simulink model "SpaceRobot"  (R2025b)
settings: Solver=ode4  StartTime=0.0  StopTime=8.5  FixedStep=0.01  RelTol=1e-5  AbsTol=1e-6
undefined symbols (not defined in the file or in its folder): d_safe, isdone_init, reward_init, Ts_agent, X, Y, Z
libraries: sm_lib x53, nesl_utility x34, rllib x1, sharedutil x1
(part 2 of 2)

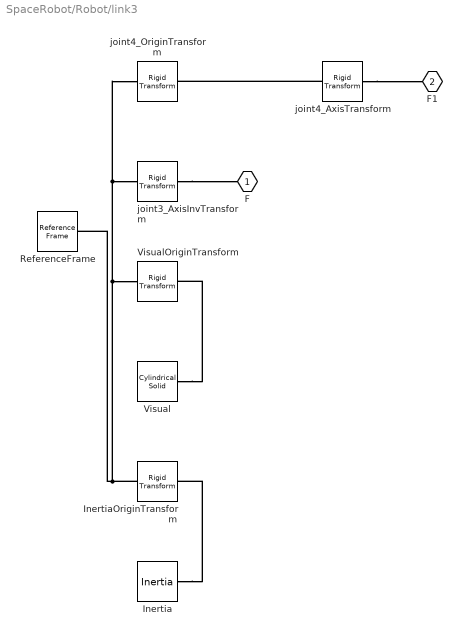
== system SpaceRobot/Robot/link3 ==
  Inertia : sm_lib/Body Elements/Inertia  InertiaType=Custom  Mass=1  MassUnits=kg  CenterOfMass=[0, 0, 0]  CenterOfMassUnits=m  MomentsOfInertia=[0.1, 0.1, 0.1]  MomentsOfInertiaUnits=kg*m^2  ProductsOfInertia=[0, 0, 0]  ProductsOfInertiaUnits=kg*m^2  GraphicType=None  MarkerShape=Inertia  MarkerSize=20  GraphicVisPropType=SimpleVisualProperties  GraphicDiffuseColor=[0.5 0.5 0.5]  GraphicOpacity=1  GraphicSpecularColor=[0.5 0.5 0.5 1.0]  GraphicAmbientColor=[0.15 0.15 0.15 1.0]  GraphicEmissiveColor=[0.0 0.0 0.0 1.0]  GraphicShininess=75
  InertiaOriginTransform : sm_lib/Frames and Transforms/Rigid Transform  RotationMethod=RotationSequence  FollAlignAxisA=+X  BaseAlignAxisA=+Y  FollAlignAxisB=+Y  BaseAlignAxisB=+Z  RotationStandardAxis=+Z  RotationAngle=0  RotationAngleUnits=deg  RotationArbitraryAxis=[0 0 1]  RotationSequenceAxes=BaseAxes  RotationSequence=XYZ  RotationSequenceAngles=[0, 0, 0]  RotationSequenceAnglesUnits=rad  RotationMatrix=[1 0 0;0 1 0;0 0 1]  Quaternion=[1 0 0 0]  TranslationMethod=Cartesian  TranslationCartesianOffset=[0.5, 0, 0]  TranslationCartesianOffsetUnits=m  TranslationStandardAxis=+Z  TranslationStandardOffset=0  TranslationStandardOffsetUnits=m  TranslationROffset=0  TranslationROffsetUnits=m  TranslationThetaOffset=0  TranslationThetaOffsetUnits=deg  TranslationZOffset=0  TranslationZOffsetUnits=m
  ReferenceFrame : sm_lib/Frames and Transforms/Reference Frame
  Visual : sm_lib/Body Elements/Cylindrical Solid  CylinderRadius=0.05  CylinderRadiusUnits=m  CylinderLength=1  CylinderLengthUnits=m  ExportEntireGeometry=off  InertiaType=Custom  BasedOnType=Density  Density=1000  DensityUnits=kg/m^3  Mass=1  MassUnits=kg  CenterOfMass=[0, 0, 0]  CenterOfMassUnits=m  MomentsOfInertia=[0.1, 0.1, 0.1]  MomentsOfInertiaUnits=kg*m^2  ProductsOfInertia=[0, 0, 0]  ProductsOfInertiaUnits=kg*m^2  GraphicType=FromGeometry  MarkerShape=Sphere  MarkerSize=10  GraphicVisPropType=SimpleVisualProperties  GraphicDiffuseColor=[0.7, 0.7, 0.7]  GraphicOpacity=1  GraphicSpecularColor=[0.5 0.5 0.5 1.0]  GraphicAmbientColor=[0.15 0.15 0.15 1.0]  GraphicEmissiveColor=[0.0 0.0 0.0 1.0]  GraphicShininess=75  DoExposeReferenceFrame=on  SerializedFrames=<Frames/>
  VisualOriginTransform : sm_lib/Frames and Transforms/Rigid Transform  RotationMethod=RotationSequence  FollAlignAxisA=+X  BaseAlignAxisA=+Y  FollAlignAxisB=+Y  BaseAlignAxisB=+Z  RotationStandardAxis=+Z  RotationAngle=0  RotationAngleUnits=deg  RotationArbitraryAxis=[0 0 1]  RotationSequenceAxes=BaseAxes  RotationSequence=XYZ  RotationSequenceAngles=[0, 1.5708, 0]  RotationSequenceAnglesUnits=rad  RotationMatrix=[1 0 0;0 1 0;0 0 1]  Quaternion=[1 0 0 0]  TranslationMethod=Cartesian  TranslationCartesianOffset=[0.5, 0, 0]  TranslationCartesianOffsetUnits=m  TranslationStandardAxis=+Z  TranslationStandardOffset=0  TranslationStandardOffsetUnits=m  TranslationROffset=0  TranslationROffsetUnits=m  TranslationThetaOffset=0  TranslationThetaOffsetUnits=deg  TranslationZOffset=0  TranslationZOffsetUnits=m
  joint3_AxisInvTransform : sm_lib/Frames and Transforms/Rigid Transform  RotationMethod=ArbitraryAxis  FollAlignAxisA=+X  BaseAlignAxisA=+Y  FollAlignAxisB=+Y  BaseAlignAxisB=+Z  RotationStandardAxis=+Z  RotationAngle=0  RotationAngleUnits=rad  RotationArbitraryAxis=[1, 0, 0]  RotationSequenceAxes=FollowerAxes  RotationSequence=XYX  RotationSequenceAngles=[0 0 0]  RotationSequenceAnglesUnits=deg  RotationMatrix=[1 0 0;0 1 0;0 0 1]  Quaternion=[1 0 0 0]  TranslationMethod=Cartesian  TranslationCartesianOffset=[0, 0, 0]  TranslationCartesianOffsetUnits=m  TranslationStandardAxis=+Z  TranslationStandardOffset=0  TranslationStandardOffsetUnits=m  TranslationROffset=0  TranslationROffsetUnits=m  TranslationThetaOffset=0  TranslationThetaOffsetUnits=deg  TranslationZOffset=0  TranslationZOffsetUnits=m
  joint4_AxisTransform : sm_lib/Frames and Transforms/Rigid Transform  RotationMethod=ArbitraryAxis  FollAlignAxisA=+X  BaseAlignAxisA=+Y  FollAlignAxisB=+Y  BaseAlignAxisB=+Z  RotationStandardAxis=+Z  RotationAngle=0  RotationAngleUnits=rad  RotationArbitraryAxis=[1, 0, 0]  RotationSequenceAxes=FollowerAxes  RotationSequence=XYX  RotationSequenceAngles=[0 0 0]  RotationSequenceAnglesUnits=deg  RotationMatrix=[1 0 0;0 1 0;0 0 1]  Quaternion=[1 0 0 0]  TranslationMethod=Cartesian  TranslationCartesianOffset=[0, 0, 0]  TranslationCartesianOffsetUnits=m  TranslationStandardAxis=+Z  TranslationStandardOffset=0  TranslationStandardOffsetUnits=m  TranslationROffset=0  TranslationROffsetUnits=m  TranslationThetaOffset=0  TranslationThetaOffsetUnits=deg  TranslationZOffset=0  TranslationZOffsetUnits=m
  joint4_OriginTransform : sm_lib/Frames and Transforms/Rigid Transform  RotationMethod=RotationSequence  FollAlignAxisA=+X  BaseAlignAxisA=+Y  FollAlignAxisB=+Y  BaseAlignAxisB=+Z  RotationStandardAxis=+Z  RotationAngle=0  RotationAngleUnits=deg  RotationArbitraryAxis=[0 0 1]  RotationSequenceAxes=BaseAxes  RotationSequence=XYZ  RotationSequenceAngles=[0, 0, 0]  RotationSequenceAnglesUnits=rad  RotationMatrix=[1 0 0;0 1 0;0 0 1]  Quaternion=[1 0 0 0]  TranslationMethod=Cartesian  TranslationCartesianOffset=[1, 0, 0]  TranslationCartesianOffsetUnits=m  TranslationStandardAxis=+Z  TranslationStandardOffset=0  TranslationStandardOffsetUnits=m  TranslationROffset=0  TranslationROffsetUnits=m  TranslationThetaOffset=0  TranslationThetaOffsetUnits=deg  TranslationZOffset=0  TranslationZOffsetUnits=m
  F : PMIOPort  Side=Left
  F1 : PMIOPort  Port=2  Side=Right
  connections:
  Inertia/RConn1 -- InertiaOriginTransform/RConn1
  ReferenceFrame/RConn1 -- InertiaOriginTransform/LConn1 -- joint3_AxisInvTransform/LConn1 -- joint4_OriginTransform/LConn1 -- VisualOriginTransform/LConn1
  Visual/RConn1 -- VisualOriginTransform/RConn1
  joint3_AxisInvTransform/RConn1 -- F/RConn1
  joint4_AxisTransform/RConn1 -- F1/RConn1
  joint4_AxisTransform/LConn1 -- joint4_OriginTransform/RConn1

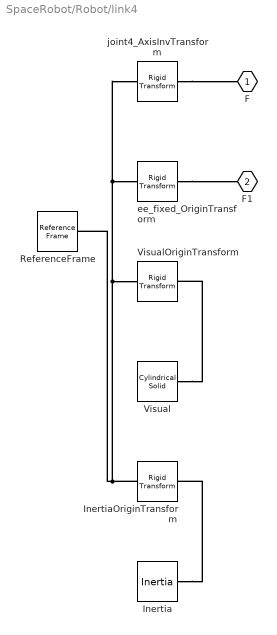
== system SpaceRobot/Robot/link4 ==
  Inertia : sm_lib/Body Elements/Inertia  InertiaType=Custom  Mass=1  MassUnits=kg  CenterOfMass=[0, 0, 0]  CenterOfMassUnits=m  MomentsOfInertia=[0.1, 0.1, 0.1]  MomentsOfInertiaUnits=kg*m^2  ProductsOfInertia=[0, 0, 0]  ProductsOfInertiaUnits=kg*m^2  GraphicType=None  MarkerShape=Inertia  MarkerSize=20  GraphicVisPropType=SimpleVisualProperties  GraphicDiffuseColor=[0.5 0.5 0.5]  GraphicOpacity=1  GraphicSpecularColor=[0.5 0.5 0.5 1.0]  GraphicAmbientColor=[0.15 0.15 0.15 1.0]  GraphicEmissiveColor=[0.0 0.0 0.0 1.0]  GraphicShininess=75
  InertiaOriginTransform : sm_lib/Frames and Transforms/Rigid Transform  RotationMethod=RotationSequence  FollAlignAxisA=+X  BaseAlignAxisA=+Y  FollAlignAxisB=+Y  BaseAlignAxisB=+Z  RotationStandardAxis=+Z  RotationAngle=0  RotationAngleUnits=deg  RotationArbitraryAxis=[0 0 1]  RotationSequenceAxes=BaseAxes  RotationSequence=XYZ  RotationSequenceAngles=[0, 0, 0]  RotationSequenceAnglesUnits=rad  RotationMatrix=[1 0 0;0 1 0;0 0 1]  Quaternion=[1 0 0 0]  TranslationMethod=Cartesian  TranslationCartesianOffset=[0.5, 0, 0]  TranslationCartesianOffsetUnits=m  TranslationStandardAxis=+Z  TranslationStandardOffset=0  TranslationStandardOffsetUnits=m  TranslationROffset=0  TranslationROffsetUnits=m  TranslationThetaOffset=0  TranslationThetaOffsetUnits=deg  TranslationZOffset=0  TranslationZOffsetUnits=m
  ReferenceFrame : sm_lib/Frames and Transforms/Reference Frame
  Visual : sm_lib/Body Elements/Cylindrical Solid  CylinderRadius=0.05  CylinderRadiusUnits=m  CylinderLength=1  CylinderLengthUnits=m  ExportEntireGeometry=off  InertiaType=Custom  BasedOnType=Density  Density=1000  DensityUnits=kg/m^3  Mass=1  MassUnits=kg  CenterOfMass=[0, 0, 0]  CenterOfMassUnits=m  MomentsOfInertia=[0.1, 0.1, 0.1]  MomentsOfInertiaUnits=kg*m^2  ProductsOfInertia=[0, 0, 0]  ProductsOfInertiaUnits=kg*m^2  GraphicType=FromGeometry  MarkerShape=Sphere  MarkerSize=10  GraphicVisPropType=SimpleVisualProperties  GraphicDiffuseColor=[0.8, 0.8, 0.8]  GraphicOpacity=1  GraphicSpecularColor=[0.5 0.5 0.5 1.0]  GraphicAmbientColor=[0.15 0.15 0.15 1.0]  GraphicEmissiveColor=[0.0 0.0 0.0 1.0]  GraphicShininess=75  DoExposeReferenceFrame=on  SerializedFrames=<Frames/>
  VisualOriginTransform : sm_lib/Frames and Transforms/Rigid Transform  RotationMethod=RotationSequence  FollAlignAxisA=+X  BaseAlignAxisA=+Y  FollAlignAxisB=+Y  BaseAlignAxisB=+Z  RotationStandardAxis=+Z  RotationAngle=0  RotationAngleUnits=deg  RotationArbitraryAxis=[0 0 1]  RotationSequenceAxes=BaseAxes  RotationSequence=XYZ  RotationSequenceAngles=[0, 1.5708, 0]  RotationSequenceAnglesUnits=rad  RotationMatrix=[1 0 0;0 1 0;0 0 1]  Quaternion=[1 0 0 0]  TranslationMethod=Cartesian  TranslationCartesianOffset=[0.5, 0, 0]  TranslationCartesianOffsetUnits=m  TranslationStandardAxis=+Z  TranslationStandardOffset=0  TranslationStandardOffsetUnits=m  TranslationROffset=0  TranslationROffsetUnits=m  TranslationThetaOffset=0  TranslationThetaOffsetUnits=deg  TranslationZOffset=0  TranslationZOffsetUnits=m
  ee_fixed_OriginTransform : sm_lib/Frames and Transforms/Rigid Transform  RotationMethod=RotationSequence  FollAlignAxisA=+X  BaseAlignAxisA=+Y  FollAlignAxisB=+Y  BaseAlignAxisB=+Z  RotationStandardAxis=+Z  RotationAngle=0  RotationAngleUnits=deg  RotationArbitraryAxis=[0 0 1]  RotationSequenceAxes=BaseAxes  RotationSequence=XYZ  RotationSequenceAngles=[0, 0, 0]  RotationSequenceAnglesUnits=rad  RotationMatrix=[1 0 0;0 1 0;0 0 1]  Quaternion=[1 0 0 0]  TranslationMethod=Cartesian  TranslationCartesianOffset=[1, 0, 0]  TranslationCartesianOffsetUnits=m  TranslationStandardAxis=+Z  TranslationStandardOffset=0  TranslationStandardOffsetUnits=m  TranslationROffset=0  TranslationROffsetUnits=m  TranslationThetaOffset=0  TranslationThetaOffsetUnits=deg  TranslationZOffset=0  TranslationZOffsetUnits=m
  joint4_AxisInvTransform : sm_lib/Frames and Transforms/Rigid Transform  RotationMethod=ArbitraryAxis  FollAlignAxisA=+X  BaseAlignAxisA=+Y  FollAlignAxisB=+Y  BaseAlignAxisB=+Z  RotationStandardAxis=+Z  RotationAngle=0  RotationAngleUnits=rad  RotationArbitraryAxis=[1, 0, 0]  RotationSequenceAxes=FollowerAxes  RotationSequence=XYX  RotationSequenceAngles=[0 0 0]  RotationSequenceAnglesUnits=deg  RotationMatrix=[1 0 0;0 1 0;0 0 1]  Quaternion=[1 0 0 0]  TranslationMethod=Cartesian  TranslationCartesianOffset=[0, 0, 0]  TranslationCartesianOffsetUnits=m  TranslationStandardAxis=+Z  TranslationStandardOffset=0  TranslationStandardOffsetUnits=m  TranslationROffset=0  TranslationROffsetUnits=m  TranslationThetaOffset=0  TranslationThetaOffsetUnits=deg  TranslationZOffset=0  TranslationZOffsetUnits=m
  F : PMIOPort  Side=Left
  F1 : PMIOPort  Port=2  Side=Right
  connections:
  Inertia/RConn1 -- InertiaOriginTransform/RConn1
  ReferenceFrame/RConn1 -- InertiaOriginTransform/LConn1 -- ee_fixed_OriginTransform/LConn1 -- joint4_AxisInvTransform/LConn1 -- VisualOriginTransform/LConn1
  Visual/RConn1 -- VisualOriginTransform/RConn1
  ee_fixed_OriginTransform/RConn1 -- F1/RConn1
  joint4_AxisInvTransform/RConn1 -- F/RConn1

== matlab function SpaceRobot/collision monitor/MATLAB Function ==
  data: q input; dmin output; isColl output
function [dmin,isColl] = collisionMonitorFcn(q)
    %#codegen
    
    coder.extrinsic('collisionCheckWrapper');
    
    % feste Outputs initialisieren
    dmin   = inf;
    isColl = false;
    
    % q auf 1x4 bringen (keine dynamische Größe!)
    nJ   = 4;
    qrow = zeros(1,nJ);
    
    L = min(numel(q), nJ);
    q_flat = reshape(q(1:L),1,[]);
    qrow(1,1:L) = q_flat;
    
    % extrinsische Kollisionsfunktion aufrufen
    dmin_ext   = dmin;
    isColl_ext = isColl;
    
    [dmin_ext, isColl_ext] = collisionCheckWrapper(qrow);
    
    dmin   = dmin_ext;
    isColl = isColl_ext;

end

== matlab function SpaceRobot/Reward/MATLAB Function ==
  data: ep input; reward output; ev input; vbase input; wbase input; tau input; tauPrev input; isDone output; e_ori input
function [reward,isDone] = rewardFcn(ep, ev, vbase, wbase, tau, tauPrev, e_ori)
    persistent prev_dist;
    if isempty(prev_dist), prev_dist = inf; end
    
    % --- Frühcheck auf Finite ---
    if any(~isfinite([ep;ev;vbase;wbase;e_ori;tau;tauPrev]))
        reward = -1; isDone = true; prev_dist = inf; return;
    end
    
    % ---- Gewichte (Startwerte) ----
    W.wp   = 150;    % EE-Position
    W.wv   = 25;     % EE-Geschwindigkeit
    W.wori = 200;    % Basis-Orientierung (P)
    W.wwb  = 8;      % Basis-Winkelgeschw. (D)
    W.wvb  = 2;      % Basis-Linear
    W.wu   = 0.02;   % Momente
    W.wd   = 0.06;   % Delta-Momente (etwas höher für Smoothness)
    
    % ---- Fortschritt ----
    dist = norm(ep);
    prog = 0;
    if isfinite(prev_dist)
        d = prev_dist - dist;
        if d>0, prog = 10*d; end
    end
    prev_dist = dist;
    
    % ---- Kosten ----
    cost  = 0;
    cost  = cost + W.wp  * (ep.'*ep);
    cost  = cost + W.wv  * (ev.'*ev);
    cost  = cost + W.wori* (e_ori.'*e_ori);  % << P auf Orientierung
    cost  = cost + W.wwb * (wbase.'*wbase);  % << D auf Orientierung
    cost  = cost + W.wvb * (vbase.'*vbase);
    cost  = cost + W.wu  * (tau.'*tau);
    cost  = cost + W.wd  * ((tau - tauPrev).'*(tau - tauPrev));
    
    % Bonus nahe Bahnpunkt
    bonus = 0.05 * exp( - (dist/0.02)^2 );
    
    reward = (prog + bonus) - cost;
    reward = reward / 500;
    
    % Abbruch
    isDone = false;
    if isnan(reward) || ~all(isfinite([ep;ev;vbase;wbase;e_ori;tau;tauPrev])) || dist>10
        isDone = true; reward = -1; prev_dist = inf;
    end
end

== matlab function SpaceRobot/Robot/Impuls Monitor/MATLAB Function ==
  data: v1 input; p_tot output; w1 input; q1 input; v2 input; w2 input; q2 input; v3 input; w3 input; q3 input; v4 input; w4 input; q4 input; v5 input; w5 input; q5 input
function p_tot = totalMomentum( ...
    v1,w1,q1, ...
    v2,w2,q2, ...
    v3,w3,q3, ...
    v4,w4,q4, ...
    v5,w5,q5)

%#codegen

    % Massen
    m = [5; 1; 1; 1; 1];

    % COM-Offsets im jeweiligen Link-Frame
    r_link = [ 0.0  0.0  0.0;   % Link 1
               0.5  0.0  0.0;   % Link 2
               0.5  0.0  0.0;   % Link 3
               0.5  0.0  0.0;   % Link 4
               0.5  0.0  0.0];  % Link 5

    % Initialisiere Gesamtimpuls
    p_tot = zeros(3,1);

    % Link 1
    p_tot = p_tot + linkMomentum(v1, w1, q1, m(1), r_link(1,:).');

    % Link 2
    p_tot = p_tot + linkMomentum(v2, w2, q2, m(2), r_link(2,:).');

    % Link 3
    p_tot = p_tot + linkMomentum(v3, w3, q3, m(3), r_link(3,:).');

    % Link 4
    p_tot = p_tot + linkMomentum(v4, w4, q4, m(4), r_link(4,:).');

    % Link 5
    p_tot = p_tot + linkMomentum(v5, w5, q5, m(5), r_link(5,:).');

end

function p = linkMomentum(v, w, q, m, r_link)
% v, w: 3x1 im World-Frame
% q: 4x1 Quaternion [w x y z], Orientierung Link relativ zu World
% r_link: 3x1 COM-Offset im Link-Frame

    % COM-Offset in World-Koordinaten drehen
    r_world = quatRotate(q, r_link);

    % COM-Geschwindigkeit
    v_com = v + cross(w, r_world);

    % Impuls dieses Links
    p = m * v_com;
end

function v_out = quatRotate(q, v_in)
% rotiert v_in (3x1) mit Quaternion q = [w x y z]

    % Normalisieren zur Sicherheit
    q = q(:) / norm(q);

    w = q(1);
    x = q(2);
    y = q(3);
    z = q(4);

    % Rotationsmatrix aus Quaternion (world <- link)
    R = [1-2*(y^2+z^2),   2*(x*y - z*w),   2*(x*z + y*w);
         2*(x*y + z*w),   1-2*(x^2+z^2),   2*(y*z - x*w);
         2*(x*z - y*w),   2*(y*z + x*w),   1-2*(x^2+y^2)];

    v_out = R * v_in(:);
end

== matlab function SpaceRobot/Robot/MATLAB Function2 ==
  data: q0 input; e_ori output; qb input
function e_ori = quatOriError(q0, qb)

    if qb(1) < 0, qb = -qb; end
    
    % ensure unit quaternions
    q0 = q0(:)/norm(q0); qb = qb(:)/norm(qb);
    
    % relative: q_err = conj(q0) * qb
    qconj = [ q0(1); -q0(2:4) ];
    qerr  = quatMultiply(qconj, qb);
    
    % keep scalar part non-negative to avoid flips
    if qerr(1) < 0
        qerr = -qerr;
    end
    
    w = qerr(1);
    v = qerr(2:4);
    nv = norm(v);
    
    if nv < 1e-12
        e_ori = [0;0;0];
    else
        theta = 2*atan2(nv, max(1e-12, w));
        u = v / nv;
        e_ori = theta * u;   % 3x1
    end
end

function q = quatMultiply(q1,q2)
    % [w x y z] * [w x y z]
    w1=q1(1); v1=q1(2:4); w2=q2(1); v2=q2(2:4);
    w  = w1*w2 - dot(v1,v2);
    v  = w1*v2 + w2*v1 + cross(v1,v2);
    q  = [w; v];
end
